simulink model "F16_6DOF_R2024b"  (R2024b)
settings: Solver=VariableStepAuto  StartTime=0.0  StopTime=10.0  RelTol=1e-3
values from neighbouring files (symbols this model uses):
  AeroBP = f16_AerodynamicData.BP    [init_F16.m]
  AeroData = f16_AerodynamicData.data    [init_F16.m]
  b = 30.0 * ft2m    (= 9.144)    [init_F16.m]    (also in trim_F16.m = sin(phi)*sin(beta) + cos(phi)*sin(alpha)*cos(beta))
  cbar = 11.32 * ft2m    (= 3.450336)    [init_F16.m]
  dP_BP = [-100, 25, 50, 100]    [init_F16.m]
  EngBP = f16_EngineData.BP    [init_F16.m]
  EngData = f16_EngineData.data.Thrust_lbs    [init_F16.m]
  Euler_0 = [0;0;0]    [init_F16.m]
  ft2m = 0.3048    [init_F16.m]
  gamma_R_SI = 1.4 * 1716.3 * R_conv    (= 401.812708631)    [init_F16.m]
  h_trop_SI = 35000 * ft2m    (= 10668)    [init_F16.m]
  He = 160.0 * slugft2_to_kgm2    (= 216.930890496)    [init_F16.m]
  I_mat = [ Ixx,  0,   -Ixz ... (first row only)    [init_F16.m]
  inv_I = inv(I_mat)    [init_F16.m]
  inv_tauT_tab = [1.0, 1.0, 0.1, 0.1]    [init_F16.m]
  lapse_SI = 0.703e-5 / ft2m    (= 2.30643044619e-05)    [init_F16.m]
  lbf2N = 4.448222    [init_F16.m]
  m = Weight / g    (= 9298.64438927)    [init_F16.m]
  omega_0 = [0;0;0]    [init_F16.m]
  P1_tab = [0, 50, 100]    [init_F16.m]
  P3_0 = 0    [init_F16.m]    (also in test_thrust_table2.m = interp1(thr_BP, P1_tab, cases(i,3)))
  Pos_0 = [0;0;-3048]    [init_F16.m]
  R0_SI = 2.377e-3 * (slug2kg / ft2m^3)    (= 1.22505555728)    [init_F16.m]
  R_ps_SI = 1715 * R_conv    (= 286.79168448)    [init_F16.m]
  S = 300.0 * (ft2m^2)    (= 27.870912)    [init_F16.m]
  T0_SI = 519.0 / 1.8    (= 288.333333333)    [init_F16.m]
  T_iso_SI = 390 / 1.8    (= 216.666666667)    [init_F16.m]
  thr_BP = [0, 77, 100]    [init_F16.m]
  V_body_0 = [131.28; 0; 0]    [init_F16.m]
  Weight = 20500.0 * lbf2N    (= 91188.551)    [init_F16.m]
  xcg = 0.35    [init_F16.m]
  xcgr = 0.35    [init_F16.m]
libraries: simulink_extras x2
(part 2 of 2)

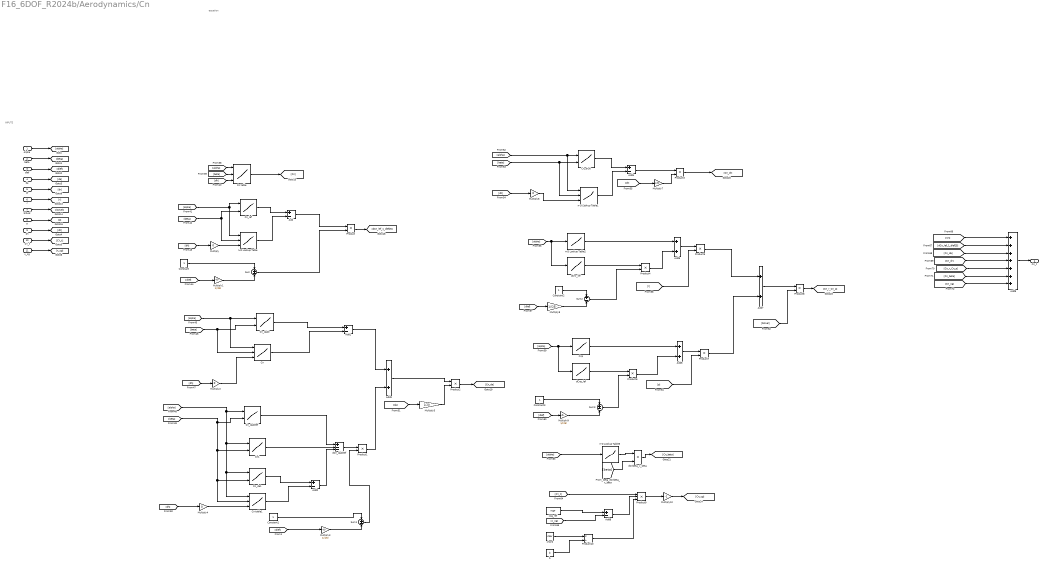
== system F16_6DOF_R2024b/Aerodynamics/Cn ==
  note: INPUTS
  note: equation
  Alpha : Inport
  beta : Inport  Port=2
  dlef : Inport  Port=3
  da : Inport  Port=4
  dr : Inport  Port=5
  r : Inport  Port=6
  bi2vel : Inport  Port=7
  p : Inport  Port=8
  dh : Inport  Port=9
  CY_t : Inport  Port=10
  x_cg : Inport  Port=11
  Add{,1..2,4,8} (5 alike) : Sum  Inputs=+-
  Add{3,5..7} (4 alike) : Sum
  Add9 : Sum  Inputs=+++++++
  Cn : Lookup_n-D  NumberOfTableDimensions=3  BreakpointsForDimension1=AeroBP.Cn.Cn.alpha  BreakpointsForDimension2=AeroBP.Cn.Cn.beta  BreakpointsForDimension3=AeroBP.Cn.Cn.dHT  Table=AeroData.Cn.Cn  ExtrapMethod=Clip  InternalRulePriority=Speed  RndMeth=Simplest
      settings: InputPortMap=u0,u1,u2
  Cn table : Lookup_n-D  NumberOfTableDimensions=3  BreakpointsForDimension1=AeroBP.Cn.Cn.alpha  BreakpointsForDimension2=AeroBP.Cn.Cn.beta  BreakpointsForDimension3=AeroBP.Cn.Cn.dHT  Table=AeroData.Cn.Cn  ExtrapMethod=Clip  InternalRulePriority=Speed  RndMeth=Simplest
      settings: InputPortMap=u0,u1,u2
  Cn table1 : Lookup_n-D  NumberOfTableDimensions=3  BreakpointsForDimension1=AeroBP.Cn.Cn.alpha  BreakpointsForDimension2=AeroBP.Cn.Cn.beta  BreakpointsForDimension3=AeroBP.Cn.Cn.dHT  Table=AeroData.Cn.Cn  ExtrapMethod=Clip  InternalRulePriority=Speed  RndMeth=Simplest
      settings: InputPortMap=u0,u1,u2
  Cn1 : Lookup_n-D  BreakpointsForDimension1=AeroBP.Cn.Cnlef.alpha  BreakpointsForDimension2=AeroBP.Cn.Cnlef.beta  BreakpointsForDimension3=[5, 7]  Table=AeroData.Cn.Cnlef  ExtrapMethod=Clip  InternalRulePriority=Speed  RndMeth=Simplest
      settings: InputPortMap=u0,u1
  Cn_da1 : Lookup_n-D  BreakpointsForDimension1=AeroBP.Cn.Cnda20.alpha  BreakpointsForDimension2=AeroBP.Cn.Cnda20.beta  BreakpointsForDimension3=[5, 7]  Table=AeroData.Cn.Cnda20  ExtrapMethod=Clip  InternalRulePriority=Speed  RndMeth=Simplest
      settings: InputPortMap=u0,u1
  Cn_da20 : Lookup_n-D  BreakpointsForDimension1=AeroBP.Cn.Cnda20.alpha  BreakpointsForDimension2=AeroBP.Cn.Cnda20.beta  BreakpointsForDimension3=[5, 7]  Table=AeroData.Cn.Cnda20  ExtrapMethod=Clip  InternalRulePriority=Speed  RndMeth=Simplest
      settings: InputPortMap=u0,u1
  Cn_da20lef : Lookup_n-D  BreakpointsForDimension1=AeroBP.Cn.Cnda20lef.alpha  BreakpointsForDimension2=AeroBP.Cn.Cnda20lef.beta  BreakpointsForDimension3=[5, 7]  Table=AeroData.Cn.Cnda20lef  ExtrapMethod=Clip  InternalRulePriority=Speed  RndMeth=Simplest
      settings: InputPortMap=u0,u1
  Cn_dr30 : Lookup_n-D  BreakpointsForDimension1=AeroBP.Cn.Cndr30.alpha  BreakpointsForDimension2=AeroBP.Cn.Cndr30.beta  BreakpointsForDimension3=[5, 7]  Table=AeroData.Cn.Cndr30  ExtrapMethod=Clip  InternalRulePriority=Speed  RndMeth=Simplest
      settings: InputPortMap=u0,u1
  Cn_lef : Lookup_n-D  BreakpointsForDimension1=AeroBP.Cn.Cnlef.alpha  BreakpointsForDimension2=AeroBP.Cn.Cnlef.beta  BreakpointsForDimension3=[5, 7]  Table=AeroData.Cn.Cnlef  ExtrapMethod=Clip  InternalRulePriority=Speed  RndMeth=Simplest
      settings: InputPortMap=u0,u1
  Cnp : Lookup_n-D  NumberOfTableDimensions=1  BreakpointsForDimension1=AeroBP.Cn.Cnp.alpha  BreakpointsForDimension3=[5, 7]  Table=AeroData.Cn.Cnp  ExtrapMethod=Clip  InternalRulePriority=Speed  RndMeth=Simplest
  Constant{,1..3} (4 alike) : Constant
  Multiply{,2,4,6} (4 alike) : Gain  Gain=0
  Multiply{1,3,8..9} (4 alike) : Gain  Gain=1/(25)
  Multiply10 : Gain  Gain=-1
  Multiply5 : Gain  Gain=1/20
  Multiply7 : Gain  Gain=1/30
  Product{,1..8} (9 alike) : Product
  Product10 : Product  Inputs=*/
  Product9 : Product  Inputs=3
  Sum{,1..3} (4 alike) : Sum  Inputs=+-
  "b " : Constant  Value=b
  chord : Constant  Value=cbar
  dCn_da20lef : Sum  Inputs=+--
  dCnbeta_x_beta : Product
  dCnp_lef : Lookup_n-D  NumberOfTableDimensions=1  BreakpointsForDimension1=AeroBP.Cn.deltaCnplef.alpha  BreakpointsForDimension3=[5, 7]  Table=AeroData.Cn.deltaCnplef  ExtrapMethod=Clip  InternalRulePriority=Speed  RndMeth=Simplest
  dCnr_lef : Lookup_n-D  NumberOfTableDimensions=1  BreakpointsForDimension1=AeroBP.Cn.deltaCnrlef.alpha  BreakpointsForDimension3=[5, 7]  Table=AeroData.Cn.deltaCnrlef  ExtrapMethod=Clip  InternalRulePriority=Speed  RndMeth=Simplest
  n-D Lookup Table : Lookup_n-D  NumberOfTableDimensions=3  BreakpointsForDimension1=AeroBP.Cn.Cn.alpha  BreakpointsForDimension2=AeroBP.Cn.Cn.beta  BreakpointsForDimension3=AeroBP.Cn.Cn.dHT  Table=AeroData.Cn.Cn  ExtrapMethod=Clip  InternalRulePriority=Speed  RndMeth=Simplest
      settings: InputPortMap=u0,u1,u2
  n-D Lookup Table1 : Lookup_n-D  NumberOfTableDimensions=3  BreakpointsForDimension1=AeroBP.Cn.Cn.alpha  BreakpointsForDimension2=AeroBP.Cn.Cn.beta  BreakpointsForDimension3=AeroBP.Cn.Cn.dHT  Table=AeroData.Cn.Cn  ExtrapMethod=Clip  InternalRulePriority=Speed  RndMeth=Simplest
      settings: InputPortMap=u0,u1,u2
  n-D Lookup Table2 : Lookup_n-D  NumberOfTableDimensions=1  BreakpointsForDimension1=AeroBP.Cn.Cnr.alpha  BreakpointsForDimension3=[5, 7]  Table=AeroData.Cn.Cnr  ExtrapMethod=Clip  InternalRulePriority=Speed  RndMeth=Simplest
  n-D Lookup Table3 : Lookup_n-D  NumberOfTableDimensions=1  BreakpointsForDimension1=AeroBP.Cn.deltaCnBeta.alpha  BreakpointsForDimension3=[5, 7]  Table=AeroData.Cn.deltaCnBeta  ExtrapMethod=Clip  InternalRulePriority=Speed  RndMeth=Simplest
  xcg_ref : Constant  Value=xcgr
  Cn_t : Outport
  wires:
  Multiply/1 -> n-D Lookup Table/3
  Add4/1 -> Product3/1
  [alpha] -> Cn table1/1, Cn_da1/1, Cn1/1, Cn_da20lef/1
  [x_cg] -> Add8/2
  Multiply8/1 -> Sum2/2
  [CY_t] -> Product9/1
  dCnr_lef/1 -> Product4/1
  [beta] -> Cn_da20/2, Cn/2
  Cn/1 -> Add1/2
  [beta] -> n-D Lookup Table/2, Cn_lef/2
  [dh] -> Multiply4/1
  [beta] -> Cn table/2
  [beta] -> n-D Lookup Table1/2, Cn_dr30/2
  Product4/1 -> Add5/2
  Multiply7/1 -> Product3/2
  Sum1/1 -> Product1/2
  [alpha] -> Cn_dr30/1, n-D Lookup Table1/1
  Constant3/1 -> Sum3/1
  Constant2/1 -> Sum2/1
  Cn_da1/1 -> Add2/1
  dCnp_lef/1 -> Product6/1
  Cn_da20/1 -> Add1/1
  Cn table1/1 -> Add2/2
  Add2/1 -> dCn_da20lef/3
  [alpha] -> Cn table/1
  [dlef] -> Multiply8/1
  Add7/1 -> Product8/1
  n-D Lookup Table/1 -> Add/2
  Cn1/1 -> dCn_da20lef/2
  Sum2/1 -> Product4/2
  [alpha] -> dCnp_lef/1, Cnp/1
  Cn table/1 -> [Cn]
  dCn_da20lef/1 -> Product1/1
  [p] -> Product7/2
  [alpha] -> Cn_lef/1, n-D Lookup Table/1
  "b "/1 -> Product10/2
  [beta] -> Cn table1/2, Cn_da1/2, Cn1/2, Cn_da20lef/2
  Product2/1 -> [Cn_da]
  Cn_da20lef/1 -> dCn_da20lef/1
  [dr] -> Multiply7/1
  Add1/1 -> Add3/1
  Product5/1 -> Add7/1
  Add5/1 -> Product5/1
  Cnp/1 -> Add6/1
  Add9/1 -> Cn_t/1
  Product7/1 -> Add7/2
  Multiply3/1 -> Sum1/2
  Constant1/1 -> Sum1/1
  [dh] -> Cn table/3
  [alpha] -> Cn_da20/1, Cn/1
  Multiply4/1 -> Cn table1/3
  [alpha] -> n-D Lookup Table3/1
  [dh] -> Multiply/1
  [da] -> Multiply5/1
  [bi2vel] -> Product8/2
  Product8/1 -> [Cn_r_Cn_p]
  Product/1 -> [dCn_lef_1_dlef25]
  [alpha] -> dCnr_lef/1, n-D Lookup Table2/1
  [dh] -> Multiply2/1
  Multiply2/1 -> Cn/3
  Multiply5/1 -> Product2/2
  Product3/1 -> [Cn_dr]
  n-D Lookup Table2/1 -> Add5/1
  Sum/1 -> Product/2
  Add/1 -> Product/1
  Multiply1/1 -> Sum/2
  Constant/1 -> Sum/1
  Cn_lef/1 -> Add/1
  [r] -> Product5/2
  [dh] -> Multiply6/1
  Product10/1 -> Product9/3
  chord/1 -> Product10/1
  Add8/1 -> Product9/2
  Product9/1 -> Multiply10/1
  xcg_ref/1 -> Add8/1
  Sum3/1 -> Product6/2
  Multiply9/1 -> Sum3/2
  Add3/1 -> Product2/1
  Product6/1 -> Add6/2
  Multiply6/1 -> n-D Lookup Table1/3
  n-D Lookup Table1/1 -> Add4/2
  Cn_dr30/1 -> Add4/1
  Add6/1 -> Product7/1
  Multiply10/1 -> [Cn_cg]
  [dlef] -> Multiply1/1
  [Cn] -> Add9/1
  [dlef] -> Multiply9/1
  Product1/1 -> Add3/2
  [dCn_lef_1_dlef25] -> Add9/2
  [Cn_r_Cn_p] -> Add9/5
  [Cn_beta] -> Add9/6
  [Cn_dr] -> Add9/4
  [Cn_da] -> Add9/3
  [Cn_cg] -> Add9/7
  da/1 -> [da]
  p/1 -> [p]
  bi2vel/1 -> [bi2vel]
  r/1 -> [r]
  beta/1 -> [beta]
  dlef/1 -> [dlef]
  Alpha/1 -> [alpha]
  dr/1 -> [dr]
  dh/1 -> [dh]
  CY_t/1 -> [CY_t]
  x_cg/1 -> [x_cg]
  [dlef] -> Multiply3/1
  n-D Lookup Table3/1 -> dCnbeta_x_beta/1
  [beta] -> dCnbeta_x_beta/2
  dCnbeta_x_beta/1 -> [Cn_beta]

== system F16_6DOF_R2024b/Propulsion/Engine Dynamics ==
  note: equation
  P_c : Inport
  P2 : Switch  Threshold=50  SaturateOnIntegerOverflow=off  InputSameDT=off
  P2_40 : Constant  Value=40
  P2_60 : Constant  Value=60
  P2_hi : Switch  Threshold=50  SaturateOnIntegerOverflow=off  InputSameDT=off
  P2_lo : Switch  Threshold=50  SaturateOnIntegerOverflow=off  InputSameDT=off
  P3_int : Integrator  InitialCondition=P3_0
  Product : Product
  RTAU : Lookup_n-D  NumberOfTableDimensions=1  BreakpointsForDimension1=dP_BP  Table=inv_tauT_tab  ExtrapMethod=Clip  InternalRulePriority=Speed  RndMeth=Simplest
  dP : Sum  Inputs=|+-
  inv_tau : Switch  Threshold=50  SaturateOnIntegerOverflow=off  InputSameDT=off
  inv_tau_5 : Constant  Value=5
  P3 : Outport
  wires:
  P_c/1 -> [P_c]
  [P_c] -> P2_hi/1
  [P3] -> P2_hi/2
  P2_60/1 -> P2_hi/3
  P2_40/1 -> P2_lo/1
  [P3] -> P2_lo/2
  [P_c] -> P2_lo/3
  P2_hi/1 -> P2/1
  [P_c] -> P2/2
  P2_lo/1 -> P2/3
  P2/1 -> dP/1
  [P3] -> dP/2
  dP/1 -> RTAU/1, Product/1
  inv_tau_5/1 -> inv_tau/1
  [P3] -> inv_tau/2
  RTAU/1 -> inv_tau/3
  inv_tau/1 -> Product/2
  Product/1 -> P3_int/1
  P3_int/1 -> [P3], P3/1
